simulink model "VCU_2023"  (Simulink 10.1)
settings: Solver=FixedStepDiscrete  StartTime=0.0  StopTime=10.0  FixedStep=0.001  RelTol=1e-3  EnableMultiTasking=on
PreLoadFcn:
  | try
  | MDL_setup;
  | catch
  | end
InitFcn:
  | EcoCoder_PreCheckLic();
undefined symbols (not defined in the file): APPS1_max, APPS1_min, APPS2_max, APPS2_min, BRK_TH, DiscIntNeverNeededParam, sigbuilder_block
libraries: CoderSF_BSW_Libs x188, simulink x28
(part 1 of 3)
settings Model: Creator=HXL  LastModifiedBy=ecuri
settings Model: SuppressorTable=|
  | <?xml version="1.0" encoding="UTF-8" standalone="yes" ?>
  | <!DOCTYPE boost_serialization>
  | <boost_serialization signature="serialization::archive" version="17">
  | <DiagnosticSuppressor class_id="0" tracking_level="0" version="6">
  | 	<Table class_id="1" tracking_level="0" version="0">
  | 		<count>4</count>
  | 		<bucket_count>8</bucket_count>
  | 		<item_version>0</item_version>
  | 		<item class_id="2" tracking_level="0" version="0">
  | 			<first class_id="3" tracking_level="0" version="6">
  | 				<Source class_id="4" tracking_level="0" version="0">
  | 					<count>1</count>
  | 					<item_version>0</item_version>
  | 					<item>VCU_2023/Main/CANbus Management/Can treatment if len=6/N_R_Dec | M_R_Dec/Extract Bits</item>
  | 				</Source>
  | 			</first>
  | 			<second class_id="5" tracking_level="0" version="6">
  | 				<SuppressedData class_id="6" tracking_level="0" version="0">
  | 					<count>2</count>
  | 					<bucket_count>8</bucket_count>
  | 					<item_version>0</item_version>
  | 					<item class_id="7" tracking_level="0" version="0">
  | 						<first class_id="8" tracking_level="0" version="6">
  | 							<ID>Simulink:DataType:WarningOverFlowDetected</ID>
  | 							<Cause>
  | 								<Source>
  | 									<count>0</count>
  | 									<item_version>0</item_version>
  | 								</Source>
  | 							</Cause>
  | 						</first>
  | 						<second class_id="9" tracking_level="0" version="6">
  | 							<Comment></Comment>
  | 							<User></User>
  | 							<LastModified class_id="10" tracking_level="0" version="0">
  | 								<ptime_date class_id="11" tracking_level="0" version="0">
  | 									<date>20160608</date>
  | 								</ptime_date>
  | 								<ptime_time_duration class_id="12" tracking_level="0" version="1">
  | 									<is_special>0</is_special>
  | 									<time_duration_hours>15</time_duration_hours>
  | 									<time_duration_minutes>43</time_duration_minutes>
  | 									<time_duration_seconds>6</time_duration_seconds>
  | 									<time_duration_fractional_seconds>0</time_duration_fractional_seconds>
  | 								</ptime_time_duration>
  | 							</LastModified>
  | 							<SuppressionType>1</SuppressionType>
  | 						</second>
  | 					</item>
  | 					<item>
  | 						<first>
  | 							<ID>SimulinkFixedPoint:util:Overflowoccurred</ID>
  | 							<Cause>
  | 								<Source>
  | 									<count>0</count>
  | 									<item_version>0</item_version>
  | 								</Source>
  | 							</Cause>
  | 						</first>
  | 						<second>
  | 							<Comment></Comment>
  | 							<User></User>
  | 							<LastModified>
  | 								<ptime_date>
  | 									<date>20160608</date>
  | 								</ptime_date>
  | 								<ptime_time_duration>
  | 									<is_special>0</is_special>
  | 									<time_duration_hours>15</time_duration_hours>
  | 									<time_duration_minutes>43</time_duration_minutes>
  | 									<time_duration_seconds>6</time_duration_seconds>
  | 									<time_duration_fractional_seconds>0</time_duration_fractional_seconds>
  | 								</ptime_time_duration>
  | 							</LastModified>
  | 							<SuppressionType>1</SuppressionType>
  | 						</second>
  | 					</item>
  | 				</SuppressedData>
  | 			</second>
  | 		</item>
  | 		<item>
  | 			<first>
  | 				<Source>
  | 					<count>1</count>
  | 					<item_version>0</item_version>
  | 					<item>VCU_2023/Main/CANbus Management/Can treatment if len=6/N_R_Dec | M_R_Dec/Extract Bits1</item>
  | 				</Source>
  | 			</first>
  | 			<second>
  | 				<SuppressedData>
  | 					<count>2</count>
  | 					<bucket_count>8</bucket_count>
  | 					<item_version>0</item_version>
  | 					<item>
  | 						<first>
  | 							<ID>Simulink:DataType:WarningOverFlowDetected</ID>
  | 							<Cause>
  | 								<Source>
  | 									<count>0</count>
  | 									<item_version>0</item_version>
  | 								</Source>
  | 							</Cause>
  | 						</first>
  | 						<second>
  | 							<Comment></Comment>
  | 							<User></User>
  | 							<LastModified>
  | 								<ptime_date>
  | 									<date>20160608</date>
  | 								</ptime_date>
  | 								<ptime_time_duration>
  | 									<is_special>0</is_special>
  | 									<time_duration_hours>15</time_duration_hours>
  | 									<time_duration_minutes>43</time_duration_minutes>
  | 									<time_duration_seconds>6</time_duration_seconds>
  | 									<time_duration_fractional_seconds>0</time_duration_fractional_seconds>
  | 								</ptime_time_duration>
  | 							</LastModified>
  | 							<SuppressionType>1</SuppressionType>
  | 						</second>
  | 					</item>
  | 					<item>
  | 						<first>
  | 							<ID>SimulinkFixedPoint:util:Overflowoccurred</ID>
  | 							<Cause>
  | 								<Source>
  | 									<count>0</count>
  | 									<item_version>0</item_version>
  | 								</Source>
  | 							</Cause>
  | 						</first>
  | 						<second>
  | 							<Comment></Comment>
  | 							<User></User>
  | 							<LastModified>
  | 								<ptime_date>
  | 									<date>20160608</date>
  | 								</ptime_date>
  | 								<ptime_time_duration>
  | 									<is_special>0</is_special>
  | 									<time_duration_hours>15</time_duration_hours>
  | 									<time_duration_minutes>43</time_duration_minutes>
  | 									<time_duration_seconds>6</time_duration_seconds>
  | 									<time_duration_fractional_seconds>0</time_duration_fractional_seconds>
  | 								</ptime_time_duration>
  | 							</LastModified>
  | 							<SuppressionType>1</SuppressionType>
  | 						</second>
  | 					</item>
  | 				</SuppressedData>
  | 			</second>
  | 		</item>
  | 		<item>
  | 			<first>
  | 				<Source>
  | 					<count>1</count>
  | 					<item_version>0</item_version>
  | 					<item>VCU_2023/Main/CANbus Management/Can treatment if len=6/N_R_Acc | M R_Acc/Extract Bits1</item>
  | 				</Source>
  | 			</first>
  | 			<second>
  | 				<SuppressedData>
  | 					<count>2</count>
  | 					<bucket_count>8</bucket_count>
  | 					<item_version>0</item_version>
  | 					<item>
  | 						<first>
  | 							<ID>Simulink:DataType:WarningOverFlowDetected</ID>
  | 							<Cause>
  | 								<Source>
  | 									<count>0</count>
  | 									<item_version>0</item_version>
  | 								</Source>
  | 							</Cause>
  | 						</first>
  | 						<second>
  | 							<Comment></Comment>
  | 							<User></User>
  | 							<LastModified>
  | 								<ptime_date>
  | 									<date>20160608</date>
  | 								</ptime_date>
  | 								<ptime_time_duration>
  | 									<is_special>0</is_special>
  | 									<time_duration_hours>15</time_duration_hours>
  | 									<time_duration_minutes>43</time_duration_minutes>
  | 									<time_duration_seconds>6</time_duration_seconds>
  | 									<time_duration_fractional_seconds>0</time_duration_fractional_seconds>
  | 								</ptime_time_duration>
  | 							</LastModified>
  | 							<SuppressionType>1</SuppressionType>
  | 						</second>
  | 					</item>
  | 					<item>
  | 						<first>
  | 							<ID>SimulinkFixedPoint:util:Overflowoccurred</ID>
  | 							<Cause>
  | 								<Source>
  | 									<count>0</count>
  | 									<item_version>0</item_version>
  | 								</Source>
  | 							</Cause>
  | 						</first>
  | 						<second>
  | 							<Comment></Comment>
  | 							<User></User>
  | 							<LastModified>
  | 								<ptime_date>
  | 									<date>20160608</date>
  | 								</ptime_date>
  | 								<ptime_time_duration>
  | 									<is_special>0</is_special>
  | 									<time_duration_hours>15</time_duration_hours>
  | 									<time_duration_minutes>43</time_duration_minutes>
  | 									<time_duration_seconds>6</time_duration_seconds>
  | 									<time_duration_fractional_seconds>0</time_duration_fractional_seconds>
  | 								</ptime_time_duration>
  | 							</LastModified>
  | 							<SuppressionType>1</SuppressionType>
  | 						</second>
  | 					</item>
  | 				</SuppressedData>
  | 			</second>
  | 		</item>
  | 		<item>
  | 			<first>
  | 				<Source>
  | 					<count>1</count>
  | 					<item_version>0</item_version>
  | 					<item>VCU_2023/Main/CANbus Management/Can treatment if len=6/N_R_Acc | M R_Acc/Extract Bits</item>
  | 				</Source>
  | 			</first>
  | 			<second>
  | 				<SuppressedData>
  | 					<count>2</count>
  | 					<bucket_count>8</bucket_count>
  | 					<item_version>0</item_version>
  | 					<item>
  | 						<first>
  | 							<ID>Simulink:DataType:WarningOverFlowDetected</ID>
  | 							<Cause>
  | 								<Source>
  | 									<count>0</count>
  | 									<item_version>0</item_version>
  | 								</Source>
  | 							</Cause>
  | 						</first>
  | 						<second>
  | 							<Comment></Comment>
  | 							<User></User>
  | 							<LastModified>
  | 								<ptime_date>
  | 									<date>20160608</date>
  | 								</ptime_date>
  | 								<ptime_time_duration>
  | 									<is_special>0</is_special>
  | 									<time_duration_hours>15</time_duration_hours>
  | 									<time_duration_minutes>43</time_duration_minutes>
  | 									<time_duration_seconds>6</time_duration_seconds>
  | 									<time_duration_fractional_seconds>0</time_duration_fractional_seconds>
  | 								</ptime_time_duration>
  | 							</LastModified>
  | 							<SuppressionType>1</SuppressionType>
  | 						</second>
  | 					</item>
  | 					<item>
  | 						<first>
  | 							<ID>SimulinkFixedPoint:util:Overflowoccurred</ID>
  | 							<Cause>
  | 								<Source>
  | 									<count>0</count>
  | 									<item_version>0</item_version>
  | 								</Source>
  | 							</Cause>
  | 						</first>
  | 						<second>
  | 							<Comment></Comment>
  | 							<User></User>
  | 							<LastModified>
  | 								<ptime_date>
  | 									<date>20160608</date>
  | 								</ptime_date>
  | 								<ptime_time_duration>
  | 									<is_special>0</is_special>
  | 									<time_duration_hours>15</time_duration_hours>
  | 									<time_duration_minutes>43</time_duration_minutes>
  | 									<time_duration_seconds>6</time_duration_seconds>
  | 									<time_duration_fractional_seconds>0</time_duration_fractional_seconds>
  | 								</ptime_time_duration>
  | 							</LastModified>
  | 							<SuppressionType>1</SuppressionType>
  | 						</second>
  | 					</item>
  | 				</SuppressedData>
  | 			</second>
  | 		</item>
  | 	</Table>
  | </DiagnosticSuppressor>
  | 
  | </boost_serialization>
  | 
  | </boost_serialization>
settings SolverCC: AutoInsertRateTranBlk=on
settings DataIOCC: ExternalInput=InputData  SaveFormat=Structure  SignalLoggingSaveFormat=ModelDataLogs  SaveOutput=off  SignalLogging=off  DSMLogging=off  SaveTime=off
settings OptimizationCC: DefaultParameterBehavior=Inlined  InlineInvariantSignals=on  EnhancedBackFolding=on  StrengthReduction=on  EnableMemcpy=off  PassReuseOutputArgsAs=Individual arguments  ExpressionDepthLimit=2147483647  EfficientFloat2IntCast=on  LifeSpan=1  SimCompilerOptimization=on  OptimizeBlockOrder=speed  DifferentSizesBufferReuse=on  EfficientTunableParamExpr=on
settings DebuggingCC: AlgebraicLoopMsg=none  ArtificialAlgebraicLoopMsg=none  SaveWithDisabledLinksMsg=none  SaveWithParameterizedLinksMsg=none  CheckSSInitialOutputMsg=off  SignalResolutionControl=TryResolveAll  BlockPriorityViolationMsg=error  MinStepSizeMsg=none  InheritedTsInSrcMsg=none  MultiTaskDSMMsg=none  MultiTaskCondExecSysMsg=none  MultiTaskRateTransMsg=warning  TasksWithSamePriorityMsg=none  SigSpecEnsureSampleTimeMsg=none  IntegerOverflowMsg=error  Int32ToFloatConvMsg=none  ParameterPrecisionLossMsg=none  ParameterTunabilityLossMsg=none  FixptConstOverflowMsg=error  FcnCallInpInsideContextMsg=warning  UnconnectedInputMsg=error  UnconnectedOutputMsg=error  UnconnectedLineMsg=error  FrameProcessingCompatibilityMsg=none  BusObjectLabelMismatch=none  RootOutportRequireBusObject=none  UnknownTsInhSupMsg=none  ModelReferenceDataLoggingMessage=none  OperatingPointInterfaceChecksumMismatchMsg=none  SFUnusedDataAndEventsDiag=none  SFUnexpectedBacktrackingDiag=none  SFInvalidInputDataAccessInChartInitDiag=none  SFNoUnconditionalDefaultTransitionDiag=none  SFTransitionOutsideNaturalParentDiag=none  SFUnreachableExecutionPathDiag=none  IntegerSaturationMsg=error
settings HardwareCC: ProdLargestAtomicInteger=Long  ProdLargestAtomicFloat=Double  ProdIntDivRoundTo=Zero  ProdEndianess=BigEndian  ProdHWDeviceType=Freescale->MPC55xx  TargetIntDivRoundTo=Zero  TargetEndianess=BigEndian  TargetHWDeviceType=Freescale->MPC55xx
settings ModelReferenceCC: UpdateModelReferenceTargets=Force  ModelReferenceNumInstancesAllowed=Single
settings SFSimCC: SFSimEcho=off  SimBuildMode=sf_make_clean  MATLABDynamicMemAlloc=off
settings RTWCC: Description=Ecotrons MPC5xxx  SystemTargetFile=MPC5644A.tlc  GenerateMakefile=off  TemplateMakefile=ert_default_tmf  RTWVerbose=off  RetainRTWFile=on  RTWCompilerOptimization=on
settings CodeAppCC: IgnoreCustomStorageClasses=off  OperatorAnnotations=on  CustomSymbolStrGlobalVar=$N$M  CustomSymbolStrType=$N$M  CustomSymbolStrFcn=$N$M  CustomSymbolStrFcnArg=$N$M  CustomSymbolStrBlkIO=$N$M  CustomSymbolStrMacro=$N$M  StateflowObjectComments=off  InternalIdentifier=Classic
settings STFCustomTargetCC: CodeReplacementLibrary=ANSI_C  UtilityFuncGeneration=Shared location  MultiwordLength=256  IncludeMdlTerminateFcn=off  CombineOutputUpdateFcns=on  SuppressErrorStatus=on  ERTCustomFileBanners=on  SupportNonFinite=off  SupportComplex=off  SupportContinuousTime=off  SupportNonInlinedSFcns=off  MATLABClassNameForMDSCustomization=Simulink.SoftwareTarget.ERTCustomization  GRTInterface=off  SystemTargetFile=MPC5644A.tlc
settings ERTTargetCC: CodeReplacementLibrary=ANSI_C  UtilityFuncGeneration=Shared location  ParMdlRefBuildCompliant=off  CompOptLevelCompliant=off  ConcurrentExecutionCompliant=off  IncludeMdlTerminateFcn=off  SuppressErrorStatus=on  SupportNonFinite=off  SupportComplex=off  RemoveResetFunc=off  ModelStepFunctionPrototypeControlCompliant=off  CPPClassGenCompliant=off  UseToolchainInfoCompliant=off  GenerateASAP2=on  InlinedParameterPlacement=NonHierarchical  ERTCustomFileTemplate=MPC5644A_file_process.tlc  ERTFilePackagingFormat=Compact  PreserveIfCondition=on  ConvertIfToSwitch=off  PreserveExternInFcnDecls=off  SuppressUnreachableDefaultCases=off
settings CustomProperty: DataType=string  Value=EV2274A
settings EnumStrPairs: String=Removed
settings ConfigComp: DVMaxProcessTime=3600  DVDisplayUnsatisfiableObjectives=on  DVModelCoverageObjectives=MCDC  DVMaxTestCaseSteps=500  DVTestSuiteOptimization=CombinedObjectives  DVDetectActiveLogic=on

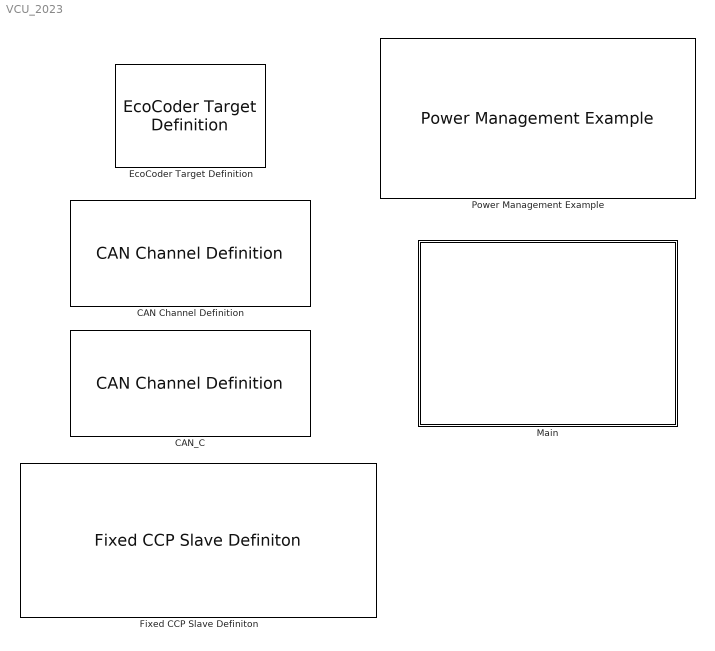
== system VCU_2023 ==
  CAN Channel Definition : CoderSF_BSW_Libs/CAN/CAN Channel Definition  channel=CAN_A  can_en=on  can_idfilter=off  can_rxextended=off  can_rxMask=hex2dec('7ff')  can_rxID=hex2dec('100')  can_baudrateIndex=500  can_txbuffer_size=30  can_rxbuffer_size=1  can_en_fd=off  nominalSamplePoint=7500  can_baudrateIndex_data=500  fastSamplePoint=7500  canfd_txbuffer_size=5  EcoCoderBlockID=C001_CANDef
  CAN_C : CoderSF_BSW_Libs/CAN/CAN Channel Definition  channel=CAN_C  can_en=on  can_idfilter=off  can_rxextended=off  can_rxMask=hex2dec('7ff')  can_rxID=hex2dec('100')  can_baudrateIndex=500  can_txbuffer_size=30  can_rxbuffer_size=1  can_en_fd=off  nominalSamplePoint=7500  can_baudrateIndex_data=500  fastSamplePoint=7500  canfd_txbuffer_size=5  EcoCoderBlockID=C001_CANDef
  EcoCoder Target Definition : CoderSF_BSW_Libs/EcoCoder Target Definition  targetECU=EV2274A  EcoCoderBlockID=T001_Target  enNoTriggerCall=on  flgBlockReduction=on  flgShowDebugDisp=off  flgDisTargetOutFIleCounter=off  flgClearAllOldFiles=on  tc275_cal_len=hex2dec('00008000')  internal_flash=[hex2dec('00020000'),hex2dec('000E0000')]  cal_rom_phy=[hex2dec('00010000'),hex2dec('00002000')]  cal_ram_wp=[hex2dec('4000F000'),hex2dec('00002000')]  cal_ram_msm=[hex2dec('40000000'),hex2dec('00002000')]  var_ram_wp=[hex2dec('40002000'),hex2dec('0000D000')]  write_back_fixed_ram=[hex2dec('40011000'),hex2dec('00001000')]  write_back_unfixed_ram=[hex2dec('40012000'),hex2dec('00001000')]  stack=[hex2dec('40013000'),hex2dec('00001000')]
      settings: AttributesFormatString=Target :%<targetECU>
  Fixed CCP Slave Definiton : CoderSF_BSW_Libs/CCP/Fixed CCP Slave Definiton  ccpType=Configurable  ccp_enSet=on  ccp_disASW=on  channel=CAN_C  stationaddressSet=hex2dec('0112')  croidSet=hex2dec('100')  dtoidSet=hex2dec('101')  daqidSet=[hex2dec('101') hex2dec('101') hex2dec('101') hex2dec('102')]  daqpidSet=[hex2dec('0') hex2dec('3C') hex2dec('78') hex2dec('0')]  daqlenSet=[hex2dec('0') hex2dec('20') hex2dec('30') hex2dec('30')]  daqperSet=[5 20 100 0]  EcoCoderBlockID=C002_CCPConf
  Main : Subsystem
  Power Management Example : CoderSF_BSW_Libs/System Management Blocks/Power Management Example  Priority=1  flgKeyFromIn=off  tKeyOffDelaySet=0.5  flgResetSWEnSet=1  tDbncKeyOffFallSet=0.1  tDbncKeyOffRiseSet=0.1  facAd2VoltSet=109/27846  uKeyOffThrSet=1  uKeyOnHystSet=1  flgCANRxLiveCheckEn=0  flgEnPwrDwnFailReset=0  flgNVMEn=on  tShtDwnWait=500  flgPwrDwnByEdgeTrigger=off  EcoCoderBlockID=PME001_Def
      settings: AttributesFormatString=Priority:%<Priority>

== system VCU_2023/Main ==
  note: Pas encore testé
  CANbus Management : Subsystem
  Data processing : Subsystem
  Main Functionalities : Subsystem
  Task Trigger : CoderSF_BSW_Libs/Task Scheduler/Task Trigger  tasktimeIndex=Task_H1ms
  Task Trigger1 : CoderSF_BSW_Libs/Task Scheduler/Task Trigger  Priority=1  tasktimeIndex=Task_L100ms  PrioritySet=1
  wires:
  Task Trigger/1 -> Main Functionalities/Trigger
  Task Trigger1/1 -> Data processing/Trigger

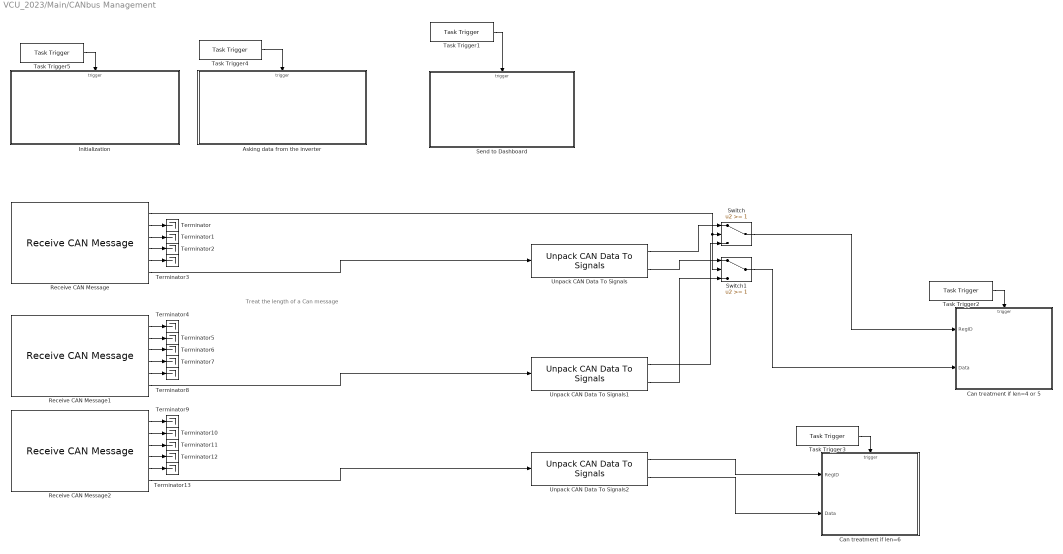
== system VCU_2023/Main/CANbus Management ==
  note: Treat the length of a Can message
  Asking data from the inverter : Subsystem
  Can treatment if len=4 or 5 : Subsystem  TreatAsAtomicUnit=on
  Can treatment if len=6 : Subsystem  TreatAsAtomicUnit=on
  Initialization : Subsystem
  Receive CAN Message : CoderSF_BSW_Libs/CAN/Receive CAN Message  channel=CAN_A  txid=hex2dec('181')  extended=off  txlen=4  tasktimeIndex=Task_L1ms
  Receive CAN Message1 : CoderSF_BSW_Libs/CAN/Receive CAN Message  channel=CAN_A  txid=hex2dec('181')  extended=off  txlen=5  tasktimeIndex=Task_L1ms
  Receive CAN Message2 : CoderSF_BSW_Libs/CAN/Receive CAN Message  channel=CAN_A  txid=hex2dec('181')  extended=off  txlen=6  tasktimeIndex=Task_L1ms
  Send to Dashboard : Subsystem  TreatAsAtomicUnit=on
  Switch : Switch  Threshold=1
  Switch1 : Switch  Threshold=1
  Task Trigger1 : CoderSF_BSW_Libs/Task Scheduler/Task Trigger  Priority=1  tasktimeIndex=Task_L100ms  PrioritySet=1
  Task Trigger2 : CoderSF_BSW_Libs/Task Scheduler/Task Trigger  Priority=1  tasktimeIndex=Task_L1ms  PrioritySet=1
  Task Trigger3 : CoderSF_BSW_Libs/Task Scheduler/Task Trigger  Priority=1  tasktimeIndex=Task_L1ms  PrioritySet=1
  Task Trigger4 : CoderSF_BSW_Libs/Task Scheduler/Task Trigger  Priority=1  tasktimeIndex=Task_H1ms  PrioritySet=1
  Task Trigger5 : CoderSF_BSW_Libs/Task Scheduler/Task Trigger  Priority=1  tasktimeIndex=Task_ini  PrioritySet=1
  Terminator{,1..13} (14 alike) : Terminator
  Unpack CAN Data To Signals : CoderSF_BSW_Libs/CAN/Unpack CAN Data To Signals  Signal={{'RegID','DATA'},[0 8],[8 32],{'uint8','uint32'},{'Intel','Intel'}}
  Unpack CAN Data To Signals1 : CoderSF_BSW_Libs/CAN/Unpack CAN Data To Signals  Signal={{'RegID','DATA'},[0 8],[8 40],{'uint8','uint32'},{'Intel','Intel'}}
  Unpack CAN Data To Signals2 : CoderSF_BSW_Libs/CAN/Unpack CAN Data To Signals  Signal={{'RegID','DATA'},[0 8],[8 48],{'uint8','uint32'},{'Intel','Intel'}}
  wires:
  Task Trigger4/1 -> Asking data from the inverter/Trigger
  Task Trigger1/1 -> Send to Dashboard/Trigger
  Unpack CAN Data To Signals/1 -> Switch/1
  Receive CAN Message/6 -> Unpack CAN Data To Signals/1
  Receive CAN Message/2 -> Terminator/1
  Receive CAN Message/3 -> Terminator1/1
  Receive CAN Message/4 -> Terminator2/1
  Receive CAN Message/5 -> Terminator3/1
  Task Trigger5/1 -> Initialization/Trigger
  Receive CAN Message/1 -> Switch1/2, Switch/2
  Receive CAN Message1/2 -> Terminator5/1
  Receive CAN Message1/3 -> Terminator6/1
  Receive CAN Message1/4 -> Terminator7/1
  Receive CAN Message1/5 -> Terminator8/1
  Receive CAN Message1/6 -> Unpack CAN Data To Signals1/1
  Unpack CAN Data To Signals1/1 -> Switch/3
  Switch/1 -> Can treatment if len=4 or 5/1(RegID)
  Switch1/1 -> Can treatment if len=4 or 5/2(Data)
  Task Trigger2/1 -> Can treatment if len=4 or 5/Trigger
  Receive CAN Message1/1 -> Terminator4/1
  Unpack CAN Data To Signals/2 -> Switch1/1
  Unpack CAN Data To Signals1/2 -> Switch1/3
  Receive CAN Message2/1 -> Terminator9/1
  Receive CAN Message2/6 -> Unpack CAN Data To Signals2/1
  Receive CAN Message2/3 -> Terminator11/1
  Receive CAN Message2/2 -> Terminator10/1
  Receive CAN Message2/4 -> Terminator12/1
  Receive CAN Message2/5 -> Terminator13/1
  Task Trigger3/1 -> Can treatment if len=6/Trigger
  Unpack CAN Data To Signals2/1 -> Can treatment if len=6/1(RegID)
  Unpack CAN Data To Signals2/2 -> Can treatment if len=6/2(Data)

== system VCU_2023/Main/Data processing ==
  Trigger : TriggerPort  TriggerType=function-call  VariantControl=Variant  PortDimensions=1
  Electrical : Subsystem
  Temperature : Subsystem

== system VCU_2023/Main/Main Functionalities ==
  Trigger : TriggerPort  TriggerType=function-call  VariantControl=Variant  PortDimensions=1
  Acceleration Pedal Position Sensors : Subsystem
      mask Display: image('C:\Users\ecuri\Desktop\BASTIE\VCU\VCU_2023\img\APPS.png'); % Use "Edit Image" on toolstrip to change.
  Brake Pressure Sensor : Subsystem
      mask Display: image('C:\Users\ecuri\Desktop\BASTIE\VCU\VCU_2023\img\BRAKE.png'); % Use "Edit Image" on toolstrip to change.
  Ready to drive : Subsystem
      mask Display: image('C:\Users\ecuri\Desktop\BASTIE\VCU\VCU_2023\img\R2D.png'); % Use "Edit Image" on toolstrip to change.
  Tractive System : Subsystem
      mask Display: image('C:\Users\ecuri\Desktop\BASTIE\VCU\VCU_2023\img\TS.png'); % Use "Edit Image" on toolstrip to change.

== system VCU_2023/Main/CANbus Management/Asking data from the inverter ==
  Trigger : TriggerPort  TriggerType=function-call  VariantControl=Variant  PortDimensions=1
  Data Type Conversion : DataTypeConversion  OutDataTypeStr=boolean
  Signal Builder : Subsystem  Tag=STV Subsys  LoadFcn=sigbuilder_block('load');  StartFcn=sigbuilder_block('start');  StopFcn=sigbuilder_block('stop');  ClipboardFcn=sigbuilder_block('clipboard');  mask(Sigbuilder block){tuvar=[0:10]}
      mask help: Simulink:masks:SigbuilderBlock_MD
      mask init:
      | if ~strcmp(get_param(bdroot(gcbh),'SimulationStatus'),'stopped') tuvar = sigbuilder_block('maskInit'); end
      settings: CopyFcn=sigbuilder_block('copy');  DeleteFcn=sigbuilder_block('delete');  ModelCloseFcn=sigbuilder_block('modelClose');  PreSaveFcn=sigbuilder_block('preSave');  PauseFcn=sigbuilder_block('pause');  ContinueFcn=sigbuilder_block('continue');  NameChangeFcn=sigbuilder_block('namechange');  OpenFcn=sigbuilder_block('open',[437.6 199.2 550.4 400 ]);  CloseFcn=sigbuilder_block('close');
      mask Display: plot(0, 0, 100, 100,[2, 2, 32, 32, 2], [68, 8, 8, 68, 68],[32, 2], [38, 38], [32, 19, 2],[53, 60, 44], [32, 17, 17, 2],[16, 16, 31, 31]);txt = getActiveGroup(gcbh);text(2, 100, txt,'verticalAlignment', 'top');
  Value separation : Subsystem
  wires:
  Signal Builder/1(Signal 1) -> Data Type Conversion/1
  Data Type Conversion/1 -> Value separation/Enable

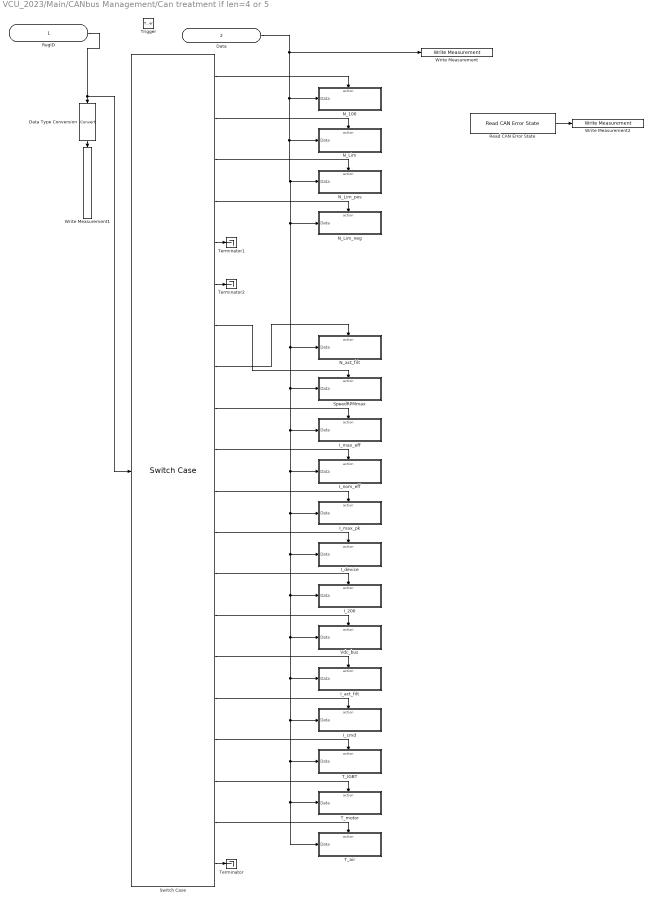
== system VCU_2023/Main/CANbus Management/Can treatment if len=4 or 5 ==
  RegID : Inport
  Data : Inport  Port=2
  Trigger : TriggerPort  TriggerType=function-call  VariantControl=Variant
  Data Type Conversion : DataTypeConversion
  I_200 : Subsystem  TreatAsAtomicUnit=on
  I_act_filt : Subsystem  TreatAsAtomicUnit=on
  I_cmd : Subsystem  TreatAsAtomicUnit=on
  I_device : Subsystem  TreatAsAtomicUnit=on
  I_max_eff : Subsystem  TreatAsAtomicUnit=on
  I_max_pk : Subsystem  TreatAsAtomicUnit=on
  I_nom_eff : Subsystem  TreatAsAtomicUnit=on
  N_100 : Subsystem  TreatAsAtomicUnit=on
  N_Lim : Subsystem  TreatAsAtomicUnit=on
  N_Lim_neg : Subsystem  TreatAsAtomicUnit=on
  N_Lim_pos : Subsystem  TreatAsAtomicUnit=on
  N_act_filt : Subsystem  TreatAsAtomicUnit=on
  Read CAN Error State : CoderSF_BSW_Libs/CAN/Read CAN Error State  channel=CAN_A
  SpeedRPMmax : Subsystem  TreatAsAtomicUnit=on
  Switch Case : SwitchCase  CaseConditions={0xc8,0x34,0x3f,0x3e,0x35,0xed,0xce,0xa8,0x4d,0x4e,0xc4,0xc6,0xd9,0xeb,0x5f,0x26,0x4a,0x49,0x4b}
  T_IGBT : Subsystem  TreatAsAtomicUnit=on
  T_air : Subsystem  TreatAsAtomicUnit=on
  T_motor : Subsystem  TreatAsAtomicUnit=on
  Terminator : Terminator
  Terminator1 : Terminator
  Terminator2 : Terminator
  Vdc_bus : Subsystem  TreatAsAtomicUnit=on
  Write Measurement : CoderSF_BSW_Libs/Calibration & Measurement/Write Measurement  variable_name=DATA  variable_value=0  variable_type=uint32  numD=1  unitStr=""  descStr=""
      settings: AttributesFormatString=type:%<variable_type> Dimensions:%<numD>
  Write Measurement1 : CoderSF_BSW_Libs/Calibration & Measurement/Write Measurement  variable_name=REGID  variable_value=0  variable_type=int16  numD=1  unitStr=""  descStr=""
      settings: AttributesFormatString=type:%<variable_type> Dimensions:%<numD>
  Write Measurement2 : CoderSF_BSW_Libs/Calibration & Measurement/Write Measurement  variable_name=stErrroaerazg  variable_value=0  variable_type=uint8  numD=1  unitStr=""  descStr=""
      settings: AttributesFormatString=type:%<variable_type> Dimensions:%<numD>
  wires:
  Switch Case/15 -> I_act_filt/Action
  Switch Case/17 -> T_IGBT/Action
  Switch Case/10 -> I_nom_eff/Action
  Switch Case/18 -> T_motor/Action
  Switch Case/13 -> I_200/Action
  Switch Case/16 -> I_cmd/Action
  Switch Case/11 -> I_max_pk/Action
  Switch Case/9 -> I_max_eff/Action
  Switch Case/14 -> Vdc_bus/Action
  Switch Case/1 -> N_100/Action
  Switch Case/4 -> N_Lim_neg/Action
  Switch Case/19 -> T_air/Action
  Switch Case/2 -> N_Lim/Action
  Switch Case/20 -> Terminator/1
  Switch Case/12 -> I_device/Action
  Switch Case/3 -> N_Lim_pos/Action
  Data Type Conversion/1 -> Write Measurement1/1
  RegID/1 -> Switch Case/1, Data Type Conversion/1
  Data/1 -> Write Measurement/1, T_air/1(Data), T_motor/1(Data), T_IGBT/1(Data), I_cmd/1(Data), I_act_filt/1(Data), Vdc_bus/1(Data), I_200/1(Data), I_device/1(Data), I_max_pk/1(Data), I_nom_eff/1(Data), I_max_eff/1(Data), SpeedRPMmax/1(Data), N_act_filt/1(Data), N_Lim_neg/1(Data), N_Lim_pos/1(Data), N_Lim/1(Data), N_100/1(Data)
  Read CAN Error State/1 -> Write Measurement2/1
  Switch Case/5 -> Terminator1/1
  Switch Case/6 -> Terminator2/1
  Switch Case/7 -> SpeedRPMmax/Action
  Switch Case/8 -> N_act_filt/Action

== system VCU_2023/Main/CANbus Management/Can treatment if len=6 ==
  RegID : Inport
  Data : Inport  Port=2
  Trigger : TriggerPort  TriggerType=function-call  VariantControl=Variant
  N_R_Acc | M R_Acc : Subsystem  TreatAsAtomicUnit=on
  N_R_Dec | M_R_Dec : Subsystem  TreatAsAtomicUnit=on
  Switch Case : SwitchCase  CaseConditions={0x35,0xed}
  Terminator : Terminator
  wires:
  Switch Case/3 -> Terminator/1
  Data/1 -> N_R_Acc | M R_Acc/1(Data), N_R_Dec | M_R_Dec/1(Data)
  Switch Case/1 -> N_R_Acc | M R_Acc/Action
  Switch Case/2 -> N_R_Dec | M_R_Dec/Action
  RegID/1 -> Switch Case/1

== system VCU_2023/Main/CANbus Management/Initialization ==
  Trigger : TriggerPort  TriggerType=function-call  VariantControl=Variant  PortDimensions=1
  Constant1 : Constant  OutDataTypeStr=boolean
  Disabling the inverter : Subsystem  Commented=on
  FRG/RUN : CoderSF_BSW_Libs/Digital I//O/Switch Output  channel=HSO02
  wires:
  Constant1/1 -> FRG/RUN/1

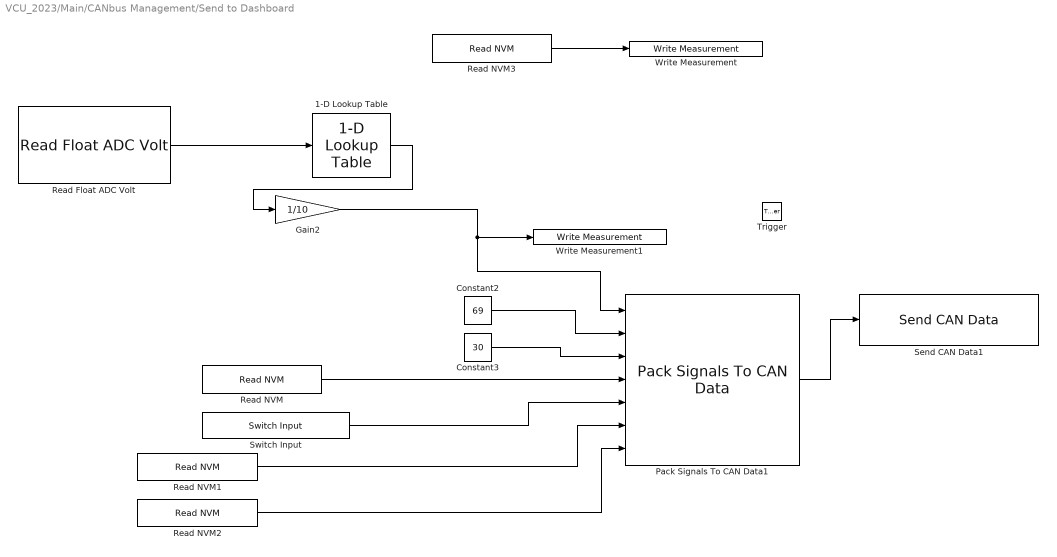
== system VCU_2023/Main/CANbus Management/Send to Dashboard ==
  Trigger : TriggerPort  TriggerType=function-call  VariantControl=Variant  PortDimensions=1
  1-D Lookup Table : CoderSF_BSW_Libs/Calibration & Measurement/1-D Lookup Table  nam=SOC  breakpoint_type=single  breakpoint_data=|  table_type=uint16  table_data=|
      breakpoint_data=|
      | [9.148916401
      | 9.635840285
      | 9.903115828
      | 10.10599429
      | 10.27061113
      | 10.40929495
      | 10.52943302
      | 10.63486361
      | 10.72797841
      | 10.81004457
      | 10.8810848
      | 10.94195341
      | 10.99707922
      | 11.04877521
      | 11.09947346
      | 11.14691464
      | 11.19124251
      | 11.23260353
      | 11.27198827
      | 11.30989032
      | 11.34851109
      | 11.3874526
      | 11.42654751
      | 11.46495999
      | 11.50120921
      | 11.53525599
      | 11.56833738
      | 11.60088018
      | 11.63218329
      | 11.66261685
      | 11.69192871
      | 11.72071681
      | 11.74878897
      | 11.77638046
      | 11.80261281
      | 11.82820664
      | 11.85751137
      | 11.8862021
      | 11.91015762
      | 11.93104465
      | 11.94984704
      | 11.96764509
      | 11.98487643
      | 12.00158425
      | 12.01806345
      | 12.03431226
      | 12.05041075
      | 12.06688244
      | 12.08321464
      | 12.10043854
      | 12.11875071
      | 12.13801533
      | 12.15845581
      | 12.178255
      | 12.19800077
      | 12.21698812
      | 12.23646291
      | 12.25546634
      | 12.27407461
      | 12.29167669
      | 12.30874131
      | 12.32538295
      | 12.34100322
      | 12.35600624
      | 12.37074328
      | 12.38506523
      | 12.3991245
      | 12.41282832
      | 12.42647057
      | 12.44007619
      | 12.45358585
      | 12.46753109
      | 12.48073355
      | 12.49411426
      | 12.5069087
      | 12.5199725
      | 12.53268034
      | 12.54539074
      | 12.55772382
      | 12.57059621
      | 12.58312348
      | 12.59544942
      | 12.60815021
      | 12.62105075
      | 12.63389833
      | 12.64687602
      | 12.66024245
      | 12.67379074
      | 12.68744713
      | 12.70154123
      | 12.71607992
      | 12.73068625
      | 12.74542514
      | 12.76078895
      | 12.77643548
      | 12.79240394
      | 12.80861387
      | 12.82499643
      | 12.84160441
      | 12.85849038
      | 12.8755599
      | 12.89256815
      | 12.90992309
      | 12.9267505
      | 12.94413739
      | 12.9610605
      | 12.97816865
      | 12.99511529
      | 13.01221545
      | 13.0290558
      | 13.04567683
      | 13.06250547
      | 13.07940342
      | 13.09628123
      | 13.11311931
      | 13.13054632
      | 13.14823906
      | 13.16647049
      | 13.18532045
      | 13.20465903
      | 13.22354217
      | 13.2419872
      | 13.25890161
      | 13.27535488
      | 13.29117581
      | 13.30693629
      | 13.32224316
      | 13.33789355
      | 13.35332499
      | 13.36858783
      | 13.38397035
      | 13.39868278
      | 13.41328735
      | 13.42742799
      | 13.4413169
      | 13.45432653
      | 13.46738568
      | 13.48050769
      | 13.49299883
      | 13.50603128
      | 13.5189436
      | 13.53231837
      | 13.54630654
      | 13.56043011
      | 13.57559703
      | 13.59100823
      | 13.60761925
      | 13.62444776
      | 13.64226923
      | 13.66092131
      | 13.67996618
      | 13.69995745
      | 13.72055645
      | 13.7417883
      | 13.763507
      | 13.78559668
      | 13.80754325
      | 13.8297083
      | 13.85188472
      | 13.87329192
      | 13.89456462
      | 13.91506045
      | 13.93487585
      | 13.95385636
      | 13.97205624
      | 13.98910303
      | 14.00517936
      | 14.01995757
      | 14.03292526
      | 14.04436994
      | 14.05354252
      | 14.06126361
      | 14.06788784
      | 14.07315504
      | 14.07799986
      | 14.08246719
      | 14.08668252
      | 14.09087421
      | 14.0947717
      | 14.09927711
      | 14.10358975
      | 14.10814705
      | 14.11299929
      | 14.1186148
      | 14.12422142
      | 14.13057656
      | 14.13698114
      | 14.14487472
      | 14.15329125
      | 14.16249672
      | 14.17312737
      | 14.1849776
      | 14.19891106
      | 14.21469493
      | 14.23323322
      | 14.25473836
      | 14.27941039
      | 14.30906477
      | 14.34290472
      | 14.38298772
      | 14.50016939]
      table_data=|
      | [0
      | 5
      | 10
      | 15
      | 20
      | 25
      | 30
      | 35
      | 40
      | 45
      | 50
      | 55
      | 60
      | 65
      | 70
      | 75
      | 80
      | 85
      | 90
      | 95
      | 100
      | 105
      | 110
      | 115
      | 120
      | 125
      | 130
      | 135
      | 140
      | 145
      | 150
      | 155
      | 160
      | 165
      | 170
      | 175
      | 180
      | 185
      | 190
      | 195
      | 200
      | 205
      | 210
      | 215
      | 220
      | 225
      | 230
      | 235
      | 240
      | 245
      | 250
      | 255
      | 260
      | 265
      | 270
      | 275
      | 280
      | 285
      | 290
      | 295
      | 300
      | 305
      | 310
      | 315
      | 320
      | 325
      | 330
      | 335
      | 340
      | 345
      | 350
      | 355
      | 360
      | 365
      | 370
      | 375
      | 380
      | 385
      | 390
      | 395
      | 400
      | 405
      | 410
      | 415
      | 420
      | 425
      | 430
      | 435
      | 440
      | 445
      | 450
      | 455
      | 460
      | 465
      | 470
      | 475
      | 480
      | 485
      | 490
      | 495
      | 500
      | 505
      | 510
      | 515
      | 520
      | 525
      | 530
      | 535
      | 540
      | 545
      | 550
      | 555
      | 560
      | 565
      | 570
      | 575
      | 580
      | 585
      | 590
      | 595
      | 600
      | 605
      | 610
      | 615
      | 620
      | 625
      | 630
      | 635
      | 640
      | 645
      | 650
      | 655
      | 660
      | 665
      | 670
      | 675
      | 680
      | 685
      | 690
      | 695
      | 700
      | 705
      | 710
      | 715
      | 720
      | 725
      | 730
      | 735
      | 740
      | 745
      | 750
      | 755
      | 760
      | 765
      | 770
      | 775
      | 780
      | 785
      | 790
      | 795
      | 800
      | 805
      | 810
      | 815
      | 820
      | 825
      | 830
      | 835
      | 840
      | 845
      | 850
      | 855
      | 860
      | 865
      | 870
      | 875
      | 880
      | 885
      | 890
      | 895
      | 900
      | 905
      | 910
      | 915
      | 920
      | 925
      | 930
      | 935
      | 940
      | 945
      | 950
      | 955
      | 960
      | 965
      | 970
      | 975
      | 980
      | 985
      | 990
      | 995
      | 1000]
  Constant2 : Constant  Value=69  OutDataTypeStr=uint8
  Constant3 : Constant  Value=30  OutDataTypeStr=uint8
  Gain2 : Gain  Gain=1/10  OutDataTypeStr=uint8
  Pack Signals To CAN Data1 : CoderSF_BSW_Libs/CAN/Pack Signals To CAN Data  Signal="{{'LVL_LV'  'LVL_HV' 'T_HV' 'APPS' 'DISP_BTN' 'TS_ON' 'R2D'},[0 8 16 24 32 40 48],[8 8 8 2 2 2 2],{'uint8' 'uint8' 'uint8' 'boolean' 'boolean' 'boolean' 'boolean'},{'Intel' 'Intel' 'Intel' 'Intel' 'Intel' 'Intel' 'Intel'}}"
      settings: AttributesFormatString=%<Parameters>
  Read Float ADC Volt : CoderSF_BSW_Libs/ADC/Read Float ADC Volt  channel=18  voltType=Custom Voltage Ratio  adType=12Bit  ratioV=(22+3.48)/3.48  voltRef=5
  Read NVM : CoderSF_BSW_Libs/Non-volatile Memory Blocks/Read NVM  variable_name=nvmAPPS_PBM  variable_type=Inherit from 'Variable definition'
  Read NVM1 : CoderSF_BSW_Libs/Non-volatile Memory Blocks/Read NVM  variable_name=nvm_TS_ON  variable_type=Inherit from 'Variable definition'
  Read NVM2 : CoderSF_BSW_Libs/Non-volatile Memory Blocks/Read NVM  variable_name=nvm_R2D  variable_type=Inherit from 'Variable definition'
  Read NVM3 : CoderSF_BSW_Libs/Non-volatile Memory Blocks/Read NVM  variable_name=nvmVdc_bus_V  variable_type=Inherit from 'Variable definition'
  Send CAN Data1 : CoderSF_BSW_Libs/CAN/Send CAN Data  channel=CAN_C  txlen=7  txid=hex2dec('38')  frametype=Standard(11-bit ID)  showerror=off
  Switch Input : CoderSF_BSW_Libs/Digital I//O/Switch Input  portNum=DI08
  Write Measurement : CoderSF_BSW_Libs/Calibration & Measurement/Write Measurement  variable_name=Tension  variable_value=0  variable_type=int16  numD=1  unitStr=""  descStr=""
      settings: AttributesFormatString=type:%<variable_type> Dimensions:%<numD>
  Write Measurement1 : CoderSF_BSW_Libs/Calibration & Measurement/Write Measurement  variable_name=LVS_PERCENT  variable_value=0  variable_type=uint8  numD=1  unitStr=""  descStr=""
      settings: AttributesFormatString=type:%<variable_type> Dimensions:%<numD>
  wires:
  Pack Signals To CAN Data1/1 -> Send CAN Data1/1
  Constant2/1 -> Pack Signals To CAN Data1/2
  Constant3/1 -> Pack Signals To CAN Data1/3
  Read NVM/1 -> Pack Signals To CAN Data1/4
  Gain2/1 -> Pack Signals To CAN Data1/1, Write Measurement1/1
  Switch Input/1 -> Pack Signals To CAN Data1/5
  Read Float ADC Volt/1 -> 1-D Lookup Table/1
  1-D Lookup Table/1 -> Gain2/1
  Read NVM1/1 -> Pack Signals To CAN Data1/6
  Read NVM2/1 -> Pack Signals To CAN Data1/7
  Read NVM3/1 -> Write Measurement/1

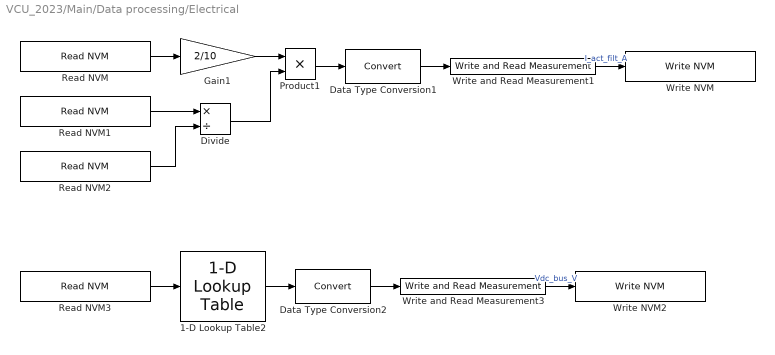
== system VCU_2023/Main/Data processing/Electrical ==
  1-D Lookup Table2 : CoderSF_BSW_Libs/Calibration & Measurement/1-D Lookup Table  nam=Vdc_bus_V  breakpoint_type=int16  breakpoint_data=[0 748 1537 2327 3117 3906 4696 5485 6275 7065 7854 8644 9434 10223 11013 11802 12592 13382 14171 14961 15751 16540 17330 18119 18909 19699 20488 21278 22067 22857 23647 24436 25226 26016 26805 27595 28384 29174 29964 30753 31543 31751]  table_type=int16  table_data=[0 25 50 75 100 125 150 175 200 225 250 275 300 325 350 375 400 425 450 475 500 525 550 575 600 625 650 675 700 725 750 775 800 825 850 875 900 925 950 975 1000 1025]
  Data Type Conversion1 : DataTypeConversion
  Data Type Conversion2 : DataTypeConversion
  Divide : Product  Inputs=*/
  Gain1 : Gain  Gain=2/10
  Product1 : Product
  Read NVM : CoderSF_BSW_Libs/Non-volatile Memory Blocks/Read NVM  variable_name=nvmI_device  variable_type=Inherit from 'Variable definition'
  Read NVM1 : CoderSF_BSW_Libs/Non-volatile Memory Blocks/Read NVM  variable_name=nvmI_act_filt  variable_type=Inherit from 'Variable definition'
  Read NVM2 : CoderSF_BSW_Libs/Non-volatile Memory Blocks/Read NVM  variable_name=nvmI_200  variable_type=Inherit from 'Variable definition'
  Read NVM3 : CoderSF_BSW_Libs/Non-volatile Memory Blocks/Read NVM  variable_name=nvmVdc_bus  variable_type=Inherit from 'Variable definition'
  Write NVM : CoderSF_BSW_Libs/Non-volatile Memory Blocks/Write NVM  variable_name=nvmI_act_filt_A  flgDef=on  variable_value=0  variable_type=int16  variable_numD=1  unitStr=A  descStr=""  EcoCoderBlockID=N001_NVMVDEF
      settings: AttributesFormatString=value:%<variable_value> type:%<variable_type> D:%<variable_numD>
  Write NVM2 : CoderSF_BSW_Libs/Non-volatile Memory Blocks/Write NVM  variable_name=nvmVdc_bus_V  flgDef=on  variable_value=0  variable_type=int16  variable_numD=1  unitStr=V  descStr=""  EcoCoderBlockID=N001_NVMVDEF
      settings: AttributesFormatString=value:%<variable_value> type:%<variable_type> D:%<variable_numD>
  Write and Read Measurement1 : CoderSF_BSW_Libs/Calibration & Measurement/Write and Read Measurement  variable_name=I_act_filt_A  variable_value=0  variable_type=int16  numD=1  unitStr=A  descStr=""
      settings: AttributesFormatString=type:%<variable_type> Dimensions:%<numD>
  Write and Read Measurement3 : CoderSF_BSW_Libs/Calibration & Measurement/Write and Read Measurement  variable_name=Vdc_bus_V  variable_value=0  variable_type=int16  numD=1  unitStr=V  descStr=""
      settings: AttributesFormatString=type:%<variable_type> Dimensions:%<numD>
  wires:
  Product1/1 -> Data Type Conversion1/1
  Divide/1 -> Product1/2
  Read NVM2/1 -> Divide/2
  Gain1/1 -> Product1/1
  Read NVM1/1 -> Divide/1
  Data Type Conversion1/1 -> Write and Read Measurement1/1
  Read NVM/1 -> Gain1/1
  Write and Read Measurement1/1 -> Write NVM/1  "I_act_filt_A"
  1-D Lookup Table2/1 -> Data Type Conversion2/1
  Write and Read Measurement3/1 -> Write NVM2/1  "Vdc_bus_V"
  Data Type Conversion2/1 -> Write and Read Measurement3/1
  Read NVM3/1 -> 1-D Lookup Table2/1

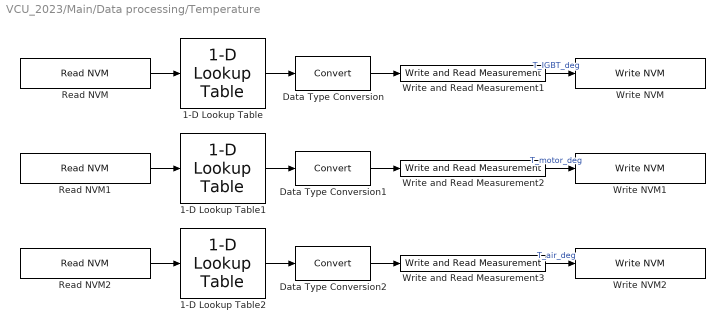
== system VCU_2023/Main/Data processing/Temperature ==
  1-D Lookup Table : CoderSF_BSW_Libs/Calibration & Measurement/1-D Lookup Table  nam=T_IGBT_conversion  breakpoint_type=int16  breakpoint_data=[16245 16308 16387 16487 16609 16759 16938 17151 17400 17688 18017 18387 18797 19247 19733 20250 20793 21357 21933 22515 23097 23671 24232 24775 25296 25792 26261 26702 27114 27497 27851 28179 28480 28757 29011 29243 29456 29650 29827]  table_type=int16  table_data=[-35 -30 -25 -20 -15 -10 -5 0 5 10 15 20 25 30 35 40 45 50 55 60 65 70 75 80 85 90 95 100 105 110 115 120 125 130 135 140 145 150 155]
  1-D Lookup Table1 : CoderSF_BSW_Libs/Calibration & Measurement/1-D Lookup Table  nam=T_motor_conversion  breakpoint_type=int16  breakpoint_data=[7414 7687 7962 8240 8520 8802 9085 9369 9654 9939 10225 10510 10795 11080 11364 11646 11927 12207 12485 12762 13036 13308 13578 13846 14111 14373 14633 14890 15144 15391 15628 15852 16061 16251 16421 16569 16692 16789 16857]  table_type=int16  table_data=[-35 -30 -25 -20 -15 -10 -5 0 5 10 15 20 25 30 35 40 45 50 55 60 65 70 75 80 85 90 95 100 105 110 115 120 125 130 135 140 145 150 155]
  1-D Lookup Table2 : CoderSF_BSW_Libs/Calibration & Measurement/1-D Lookup Table  nam=T_air_conversion  breakpoint_type=int16  breakpoint_data=[8516 8785 9054 9322 9590 9857 10122 10386 10647 10907 11163 11418 11669 11917 12163 12404 12643 12878 13109 13337 13561 13781 13998 14210 14419 14624 14825 15022 15215]  table_type=int16  table_data=[-35 -30 -25 -20 -15 -10 -5 0 5 10 15 20 25 30 35 40 45 50 55 60 65 70 75 80 85 90 95 100 105]
  Data Type Conversion : DataTypeConversion
  Data Type Conversion1 : DataTypeConversion
  Data Type Conversion2 : DataTypeConversion
  Read NVM : CoderSF_BSW_Libs/Non-volatile Memory Blocks/Read NVM  variable_name=nvmT_IGBT  variable_type=Inherit from 'Variable definition'
  Read NVM1 : CoderSF_BSW_Libs/Non-volatile Memory Blocks/Read NVM  variable_name=nvmT_motor  variable_type=Inherit from 'Variable definition'
  Read NVM2 : CoderSF_BSW_Libs/Non-volatile Memory Blocks/Read NVM  variable_name=nvmT_air  variable_type=Inherit from 'Variable definition'
  Write NVM : CoderSF_BSW_Libs/Non-volatile Memory Blocks/Write NVM  variable_name=nvmT_IGBT_deg  flgDef=on  variable_value=0  variable_type=int16  variable_numD=1  unitStr=°C  descStr=""  EcoCoderBlockID=N001_NVMVDEF
      settings: AttributesFormatString=value:%<variable_value> type:%<variable_type> D:%<variable_numD>
  Write NVM1 : CoderSF_BSW_Libs/Non-volatile Memory Blocks/Write NVM  variable_name=nvmT_motor_deg  flgDef=on  variable_value=0  variable_type=int16  variable_numD=1  unitStr=°C  descStr=""  EcoCoderBlockID=N001_NVMVDEF
      settings: AttributesFormatString=value:%<variable_value> type:%<variable_type> D:%<variable_numD>
  Write NVM2 : CoderSF_BSW_Libs/Non-volatile Memory Blocks/Write NVM  variable_name=nvmT_air_deg  flgDef=on  variable_value=0  variable_type=int16  variable_numD=1  unitStr=°C  descStr=""  EcoCoderBlockID=N001_NVMVDEF
      settings: AttributesFormatString=value:%<variable_value> type:%<variable_type> D:%<variable_numD>
  Write and Read Measurement1 : CoderSF_BSW_Libs/Calibration & Measurement/Write and Read Measurement  variable_name=T_IGBT_deg  variable_value=0  variable_type=int16  numD=1  unitStr=°C  descStr=""
      settings: AttributesFormatString=type:%<variable_type> Dimensions:%<numD>
  Write and Read Measurement2 : CoderSF_BSW_Libs/Calibration & Measurement/Write and Read Measurement  variable_name=T_motor_deg  variable_value=0  variable_type=int16  numD=1  unitStr=°C  descStr=""
      settings: AttributesFormatString=type:%<variable_type> Dimensions:%<numD>
  Write and Read Measurement3 : CoderSF_BSW_Libs/Calibration & Measurement/Write and Read Measurement  variable_name=T_air_deg  variable_value=0  variable_type=int16  numD=1  unitStr=°C  descStr=""
      settings: AttributesFormatString=type:%<variable_type> Dimensions:%<numD>
  wires:
  Write and Read Measurement1/1 -> Write NVM/1  "T_IGBT_deg"
  Read NVM/1 -> 1-D Lookup Table/1
  Data Type Conversion/1 -> Write and Read Measurement1/1
  1-D Lookup Table/1 -> Data Type Conversion/1
  Data Type Conversion1/1 -> Write and Read Measurement2/1
  1-D Lookup Table1/1 -> Data Type Conversion1/1
  Read NVM1/1 -> 1-D Lookup Table1/1
  Write and Read Measurement2/1 -> Write NVM1/1  "T_motor_deg"
  Data Type Conversion2/1 -> Write and Read Measurement3/1
  1-D Lookup Table2/1 -> Data Type Conversion2/1
  Read NVM2/1 -> 1-D Lookup Table2/1
  Write and Read Measurement3/1 -> Write NVM2/1  "T_air_deg"

== system VCU_2023/Main/Main Functionalities/Acceleration Pedal Position Sensors ==
  APPS reading and calibration : Subsystem
      mask Display: image('C:\Users\ecuri\Desktop\BASTIE\VCU\VCU_2023\img\RnC.png'); % Use "Edit Image" on toolstrip to change.
  Check APPS Implausibility : Subsystem
      mask Display: image('C:\Users\ecuri\Desktop\BASTIE\VCU\VCU_2023\img\APPS_PBM.png'); % Use "Edit Image" on toolstrip to change.
  Send Torque Command : Subsystem
      mask Display: image('C:\Users\ecuri\Desktop\BASTIE\VCU\VCU_2023\img\TORQUE.png'); % Use "Edit Image" on toolstrip to change.
  wires:
  APPS reading and calibration/1(APPS 1) -> Check APPS Implausibility/1(APPS 1), Send Torque Command/1(APPS 1)  "APPS 1"
  APPS reading and calibration/2(APPS 2) -> Check APPS Implausibility/2(APPS 2), Send Torque Command/2(APPS 2)  "APPS 2"

== system VCU_2023/Main/Main Functionalities/Brake Pressure Sensor ==
  Brake Light : CoderSF_BSW_Libs/Digital I//O/Switch Output  channel=LSO07
  Brake Pressure : CoderSF_BSW_Libs/ADC/Read ADC Value  channel=15
  Compare To Constant2 : simulink/Logic and Bit Operations/Compare To Constant  relop=>=  const=BRK_TH  OutDataTypeStr=boolean
  Data Type Conversion3 : DataTypeConversion  OutDataTypeStr=int16
  Write NVM3 : CoderSF_BSW_Libs/Non-volatile Memory Blocks/Write NVM  variable_name=nvmBRK_TH  flgDef=on  variable_value=0  variable_type=int16  variable_numD=1  unitStr=""  descStr=""  EcoCoderBlockID=N001_NVMVDEF
      settings: AttributesFormatString=value:%<variable_value> type:%<variable_type> D:%<variable_numD>
  Write and Read Measurement2 : CoderSF_BSW_Libs/Calibration & Measurement/Write and Read Measurement  variable_name=BRK_PRESSURE  variable_value=0  variable_type=uint16  numD=1  unitStr=""  descStr=""
      settings: AttributesFormatString=type:%<variable_type> Dimensions:%<numD>
  ecocoder_calibration2 : CoderSF_BSW_Libs/Calibration & Measurement/Read Calibration  variable_name=BRK_TH  variable_value=90  variable_type=int16  variable_min=[]  variable_max=[]  unitStr=""  descStr=""
      settings: AttributesFormatString=value:%<variable_value> type:%<variable_type> max:%<variable_max> Min:%<variable_min>
  tag scope: BRAKE_ON=global
  wires:
  Write and Read Measurement2/1 -> Data Type Conversion3/1  "BRK_PRESSURE"
  Data Type Conversion3/1 -> Compare To Constant2/1
  ecocoder_calibration2/1 -> Write NVM3/1
  Brake Pressure/1 -> Write and Read Measurement2/1
  Compare To Constant2/1 -> Brake Light/1, [BRAKE_ON]

== system VCU_2023/Main/Main Functionalities/Ready to drive ==
  Logical Operator : Logic  Operator=OR  Inputs=3  IconShape=distinctive  AllPortsSameDT=off  OutDataTypeStr=boolean
  Logical Operator1 : Logic  Inputs=3  IconShape=distinctive  AllPortsSameDT=off  OutDataTypeStr=boolean
  Logical Operator2 : Logic  Operator=NOT  Inputs=1  IconShape=distinctive  AllPortsSameDT=off  OutDataTypeStr=boolean
  Logical Operator3 : Logic  Operator=NOT  Inputs=1  IconShape=distinctive  AllPortsSameDT=off  OutDataTypeStr=boolean
  Logical Operator4 : Logic  Operator=NOT  Inputs=1  IconShape=distinctive  AllPortsSameDT=off  OutDataTypeStr=boolean
  Subsystem : Subsystem
      mask Display: image('C:\Users\ecuri\Desktop\BASTIE\VCU\VCU_2023\img\R2D_ACT_SEQ.png'); % Use "Edit Image" on toolstrip to change.
  Subsystem1 : Subsystem
      mask Display: image('C:\Users\ecuri\Desktop\BASTIE\VCU\VCU_2023\img\ENTER_R2D.png'); % Use "Edit Image" on toolstrip to change.
  wires:
  [APPS_PBM] -> Logical Operator3/1
  [TS_ON] -> Logical Operator1/1, Logical Operator2/1
  Logical Operator1/1 -> Logical Operator/3, Subsystem1/2(Exit)
  Logical Operator/1 -> Subsystem1/1(Trigger)
  Subsystem/1(R2D_ASKED) -> Logical Operator1/3
  Logical Operator3/1 -> Logical Operator4/1, Logical Operator1/2
  Logical Operator2/1 -> Logical Operator/1
  Logical Operator4/1 -> Logical Operator/2
